simulink library "engine_mgmt_lib"  (R2025a)
settings: Solver=VariableStepAuto  StartTime=0.0  StopTime=10.0  RelTol=1e-3
undefined symbols (not defined in the file): cmdEngSpeed
libraries: simulink x1
Description:
  | Copyright 2023-2025 The MathWorks, Inc.
settings Model: Creator=smiller  LastModifiedBy=smiller
settings OptimizationCC: ReuseModelBlockBuffer=off
settings RTWCC: GPUComputeCapability=3.5

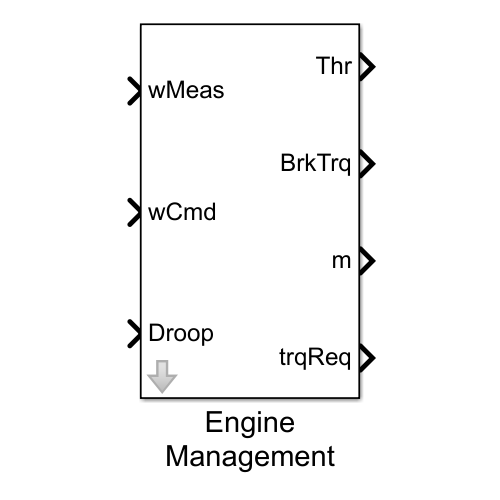
[thumbnail: Simulink's stored preview of the top-level diagram]
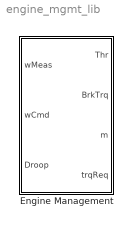
== system engine_mgmt_lib ==
  Engine Management : Subsystem  mask{kp_thr=10, ki_thr=0, kp_brk=5, ki_brk=0, engine_trq=0, engine_spd=0, w0_engine=cmdEngSpeed}
      mask prompts: kp_thr "Kp, Throttle"; ki_thr "Ki, Throttle"; kp_brk "Kp, Brake"; ki_brk "Ki, Brake"; engine_trq "Engine Curve, torque"; engine_spd "Engine Curve, Speed"; w0_engine "Initial Engine Speed"
      mask TypeOptions kp_thr:
      | Control
      | Torque Request/kp_thr
      mask TypeOptions ki_thr:
      | Control
      | Torque Request/ki_thr
      mask TypeOptions kp_brk:
      | Control
      | Torque Request/kp_brk
      mask TypeOptions ki_brk:
      | Control
      | Torque Request/ki_brk

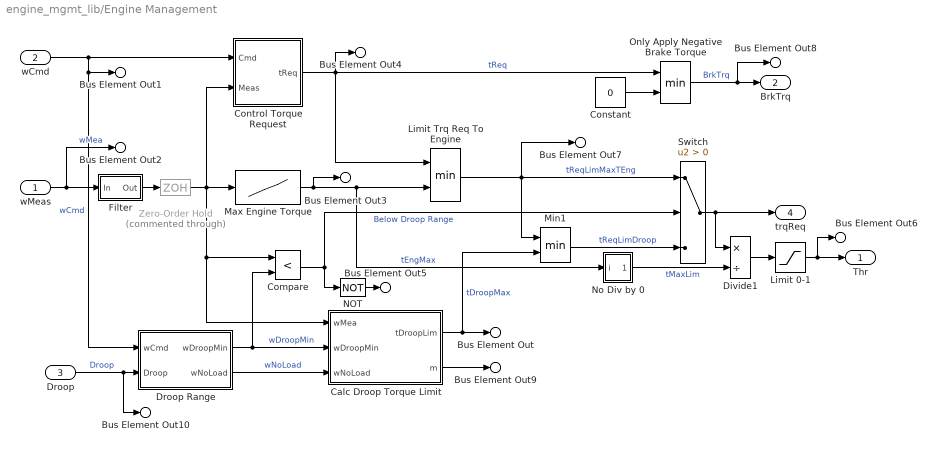
== system engine_mgmt_lib/Engine Management ==
  wMeas : Inport
  wCmd : Inport  Port=2
  Droop : Inport  Port=3
  Calc Droop Torque Limit : Subsystem
  Compare : RelationalOperator  Operator=<  OutDataTypeStr=boolean  ZeroCross=off  RndMeth=Simplest  InputSameDT=off
  Constant : Constant  Value=0
  Control Torque Request : Subsystem  mask{kp_thr=kp_thr, ki_thr=ki_thr, kp_brk=kp_brk, ki_brk=ki_brk}
      mask prompts: kp_thr "Kp, Throttle"; ki_thr "Ki, Throttle"; kp_brk "Kp, Brake"; ki_brk "Ki, Brake"
  Divide1 : Product  Inputs=*/
  Droop Range : Subsystem
  Filter : Subsystem  mask(First-order lag supporting vector signals){b=0.01, x_initial=w0_engine}
      mask prompts: b "Filter time constant"; x_initial "Initial output"
      mask help: Models a lag of the form 1/(b*s+1) where s is the Laplace operator.
  Limit 0-1 : Saturate  UpperLimit=1  LowerLimit=0  ZeroCross=off
  Limit Trq Req To Engine : MinMax  Inputs=2
  Max Engine Torque : Lookup_n-D  NumberOfTableDimensions=1  BreakpointsForDimension1=engine_spd  Table=engine_trq  InternalRulePriority=Speed  RndMeth=Simplest
  Min1 : MinMax  Inputs=2
  NOT : Logic  Operator=NOT  AllPortsSameDT=off  OutDataTypeStr=boolean
  No Div by 0 : Subsystem
  Only Apply Negative Brake Torque : MinMax  Inputs=2  ZeroCross=off
  Switch : Switch  Criteria=u2 > Threshold  ZeroCross=off  SaturateOnIntegerOverflow=off  InputSameDT=off
  Zero-Order Hold : ZeroOrderHold  Commented=through  SampleTime=0.05
  Thr : Outport  VectorParamsAs1DForOutWhenUnconnected=off
  BrkTrq : Outport  Port=2  VectorParamsAs1DForOutWhenUnconnected=off
  Bus Element Out : Outport  Port=3  PortName=m  Element=tDroopLim
  Bus Element Out1 : Outport  Port=3  PortName=m  Element=wCmd
  Bus Element Out2 : Outport  Port=3  PortName=m  Element=wMea
  Bus Element Out3 : Outport  Port=3  PortName=m  Element=tEngMax
  Bus Element Out4 : Outport  Port=3  PortName=m  Element=tReq
  Bus Element Out5 : Outport  Port=3  PortName=m  Element=inDroop
  Bus Element Out6 : Outport  Port=3  PortName=m  Element=Thr
  Bus Element Out7 : Outport  Port=3  PortName=m  Element=tReqLim
  Bus Element Out8 : Outport  Port=3  PortName=m  Element=brkTrq
  Bus Element Out9 : Outport  Port=3  PortName=m  Element=CalcDroopLim
  Bus Element Out10 : Outport  Port=3  PortName=m  Element=droop
  trqReq : Outport  Port=4  VectorParamsAs1DForOutWhenUnconnected=off
  wires:
  wMeas/1 -> Filter/1(In), Bus Element Out2/1  "wMea"
  Only Apply Negative Brake Torque/1 -> Bus Element Out8/1, BrkTrq/1  "BrkTrq"
  Droop/1 -> Bus Element Out10/1, Droop Range/2(Droop)  "Droop"
  No Div by 0/1(o) -> Divide1/2  "tMaxLim"
  Droop Range/2(wNoLoad) -> Calc Droop Torque Limit/3(wNoLoad)  "wNoLoad"
  Divide1/1 -> Limit 0-1/1
  Calc Droop Torque Limit/1(tDroopLim) -> Bus Element Out/1, Min1/2  "tDroopMax"
  Compare/1 -> Switch/2, NOT/1  "Below Droop Range"
  Control Torque Request/1(tReq) -> Bus Element Out4/1, Only Apply Negative Brake Torque/1, Limit Trq Req To Engine/1  "tReq"
  Min1/1 -> Switch/3  "tReqLimDroop"
  Limit Trq Req To Engine/1 -> Switch/1, Bus Element Out7/1, Min1/1  "tReqLimMaxTEng"
  wCmd/1 -> Bus Element Out1/1, Droop Range/1(wCmd), Control Torque Request/1(Cmd)  "wCmd"
  Droop Range/1(wDroopMin) -> Calc Droop Torque Limit/2(wDroopMin), Compare/2  "wDroopMin"
  Max Engine Torque/1 -> Bus Element Out3/1, Limit Trq Req To Engine/2, No Div by 0/1(i)  "tEngMax"
  Limit 0-1/1 -> Thr/1, Bus Element Out6/1
  NOT/1 -> Bus Element Out5/1
  Switch/1 -> trqReq/1, Divide1/1
  Filter/1(Out) -> Zero-Order Hold/1
  Zero-Order Hold/1 -> Calc Droop Torque Limit/1(wMea), Compare/1, Control Torque Request/2(Meas), Max Engine Torque/1
  Constant/1 -> Only Apply Negative Brake Torque/2
  Calc Droop Torque Limit/2(m) -> Bus Element Out9/1

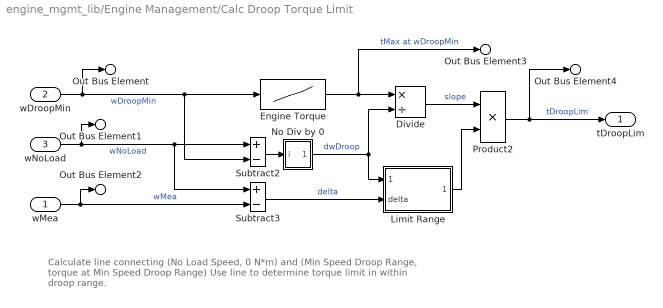
== system engine_mgmt_lib/Engine Management/Calc Droop Torque Limit ==
  note: Calculate line connecting (No Load Speed, 0 N*m) and
      | (Min Speed Droop Range, torque at Min Speed Droop Range)
      | Use line to determine torque limit in within droop range.
  wMea : Inport
  wDroopMin : Inport  Port=2
  wNoLoad : Inport  Port=3
  Divide : Product  Inputs=*/
  Engine Torque : Lookup_n-D  NumberOfTableDimensions=1  BreakpointsForDimension1=engine_spd  Table=engine_trq  InternalRulePriority=Speed  RndMeth=Simplest
  Limit Range : Subsystem
  No Div by 0 : Subsystem
  Product2 : Product
  Subtract2 : Sum  Inputs=+-
  Subtract3 : Sum  Inputs=+-
  tDroopLim : Outport
  Out Bus Element : Outport  Port=2  PortName=m  Element=wDroopMin
  Out Bus Element1 : Outport  Port=2  PortName=m  Element=wNoLoad
  Out Bus Element2 : Outport  Port=2  PortName=m  Element=wMea
  Out Bus Element3 : Outport  Port=2  PortName=m  Element=tMaxAtwDroopMin
  Out Bus Element4 : Outport  Port=2  PortName=m  Element=tDroopLim
  wires:
  Engine Torque/1 -> Divide/1, Out Bus Element3/1  "tMax at wDroopMin"
  Product2/1 -> Out Bus Element4/1, tDroopLim/1  "tDroopLim"
  Subtract2/1 -> No Div by 0/1(i)
  wDroopMin/1 -> Engine Torque/1, Subtract2/2, Out Bus Element/1  "wDroopMin"
  wMea/1 -> Out Bus Element2/1, Subtract3/2  "wMea"
  Divide/1 -> Product2/1  "slope"
  wNoLoad/1 -> Subtract3/1, Subtract2/1, Out Bus Element1/1  "wNoLoad"
  No Div by 0/1(o) -> Divide/2, Limit Range/1(dwDroop)  "dwDroop"
  Subtract3/1 -> Limit Range/2(delta)  "delta"
  Limit Range/1(wDelta) -> Product2/2

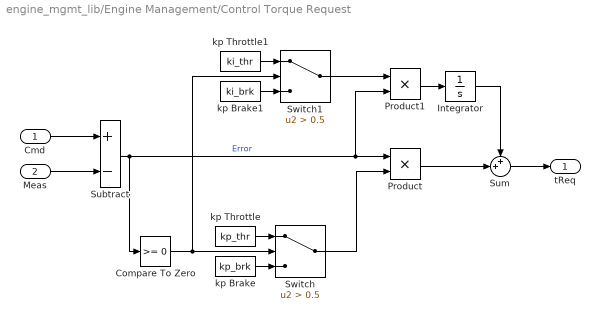
== system engine_mgmt_lib/Engine Management/Control Torque Request ==
  Cmd : Inport
  Meas : Inport  Port=2
  Compare To Zero : simulink/Logic and Bit Operations/Compare To Zero  relop=>=  OutDataTypeStr=boolean  ZeroCross=off
  Integrator : Integrator
  Product : Product
  Product1 : Product
  Subtract : Sum  Inputs=+-
  Sum : Sum  Inputs=++|
  Switch : Switch  Criteria=u2 > Threshold  Threshold=0.5  ZeroCross=off  SaturateOnIntegerOverflow=off  InputSameDT=off
  Switch1 : Switch  Criteria=u2 > Threshold  Threshold=0.5  ZeroCross=off  SaturateOnIntegerOverflow=off  InputSameDT=off
  kp Brake : Constant  Value=kp_brk
  kp Brake1 : Constant  Value=ki_brk
  kp Throttle : Constant  Value=kp_thr
  kp Throttle1 : Constant  Value=ki_thr
  tReq : Outport
  wires:
  Product1/1 -> Integrator/1
  Integrator/1 -> Sum/1
  Cmd/1 -> Subtract/1
  Meas/1 -> Subtract/2
  Sum/1 -> tReq/1
  kp Throttle/1 -> Switch/1
  kp Brake/1 -> Switch/3
  Switch/1 -> Product/2
  Compare To Zero/1 -> Switch1/2, Switch/2
  Product/1 -> Sum/2
  Subtract/1 -> Product/1, Product1/2, Compare To Zero/1  "Error"
  kp Brake1/1 -> Switch1/3
  kp Throttle1/1 -> Switch1/1
  Switch1/1 -> Product1/1

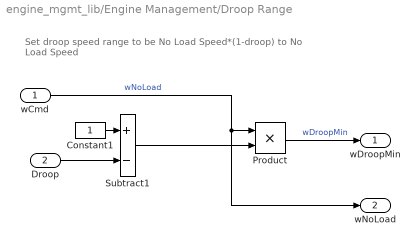
== system engine_mgmt_lib/Engine Management/Droop Range ==
  note: Set droop speed range to be
      |     No Load Speed*(1-droop)   to    No Load Speed
  wCmd : Inport
  Droop : Inport  Port=2
  Constant1 : Constant
  Product : Product
  Subtract1 : Sum  Inputs=+-
  wDroopMin : Outport
  wNoLoad : Outport  Port=2
  wires:
  Constant1/1 -> Subtract1/1
  Droop/1 -> Subtract1/2
  Product/1 -> wDroopMin/1  "wDroopMin"
  wCmd/1 -> wNoLoad/1, Product/1  "wNoLoad"
  Subtract1/1 -> Product/2

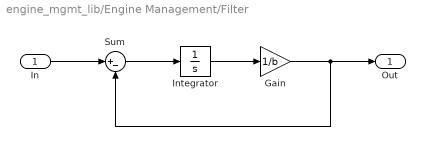
== system engine_mgmt_lib/Engine Management/Filter ==
  In : Inport
  Gain : Gain  Gain=1/b
  Integrator : Integrator  InitialCondition=x_initial*b
  Sum : Sum  Inputs=|+-  InputSameDT=on  SaturateOnIntegerOverflow=on  OutDataTypeStr=Inherit: Same as first input
  Out : Outport  VectorParamsAs1DForOutWhenUnconnected=off
  wires:
  Sum/1 -> Integrator/1
  In/1 -> Sum/1
  Integrator/1 -> Gain/1
  Gain/1 -> Sum/2, Out/1

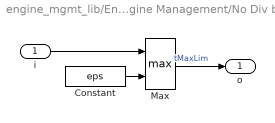
== system engine_mgmt_lib/Engine Management/No Div by 0 ==
  i : Inport
  Constant : Constant  Value=eps
  Max : MinMax  Function=max  Inputs=2
  o : Outport
  wires:
  Constant/1 -> Max/2
  i/1 -> Max/1
  Max/1 -> o/1  "tMaxLim"

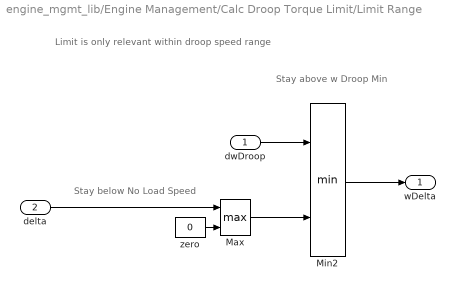
== system engine_mgmt_lib/Engine Management/Calc Droop Torque Limit/Limit Range ==
  note: Limit is only relevant within droop speed range
  note: Stay above
      | w Droop Min
  note: Stay below No Load Speed
  dwDroop : Inport
  delta : Inport  Port=2
  Max : MinMax  Function=max  Inputs=2
  Min2 : MinMax  Inputs=2
  zero : Constant  Value=0
  wDelta : Outport
  wires:
  dwDroop/1 -> Min2/1
  Max/1 -> Min2/2
  zero/1 -> Max/2
  Min2/1 -> wDelta/1
  delta/1 -> Max/1

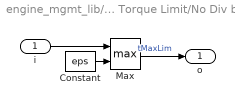
== system engine_mgmt_lib/Engine Management/Calc Droop Torque Limit/No Div by 0 ==
  i : Inport
  Constant : Constant  Value=eps
  Max : MinMax  Function=max  Inputs=2
  o : Outport
  wires:
  Constant/1 -> Max/2
  i/1 -> Max/1
  Max/1 -> o/1  "tMaxLim"
